simulink model "VFD1"  (R2023b)
settings: Solver=VariableStepAuto  StartTime=0.0  StopTime=6  RelTol=1e-3
libraries: spsACVoltageSourceLib x3, spsSeriesRLCBranchLib x2, spsUniversalBridgeLib x2, spsVoltageMeasurementLib x2, spsAsynchronousMachineSIUnitsLib x1, spsCurrentMeasurementLib x1, spsGroundLib x1, spsIGBTDiodeLib x1, spsPWMGenerator2LevelLib x1, spsRMSLib x1, sps_lib x1
settings Model: Creator=LAB203  LastModifiedBy=LAB203

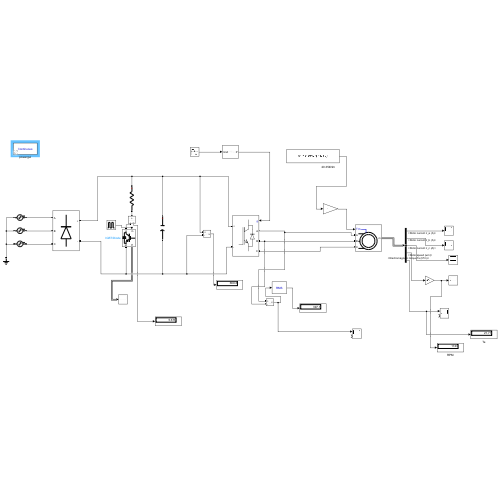
[thumbnail: Simulink's stored preview of the top-level diagram]
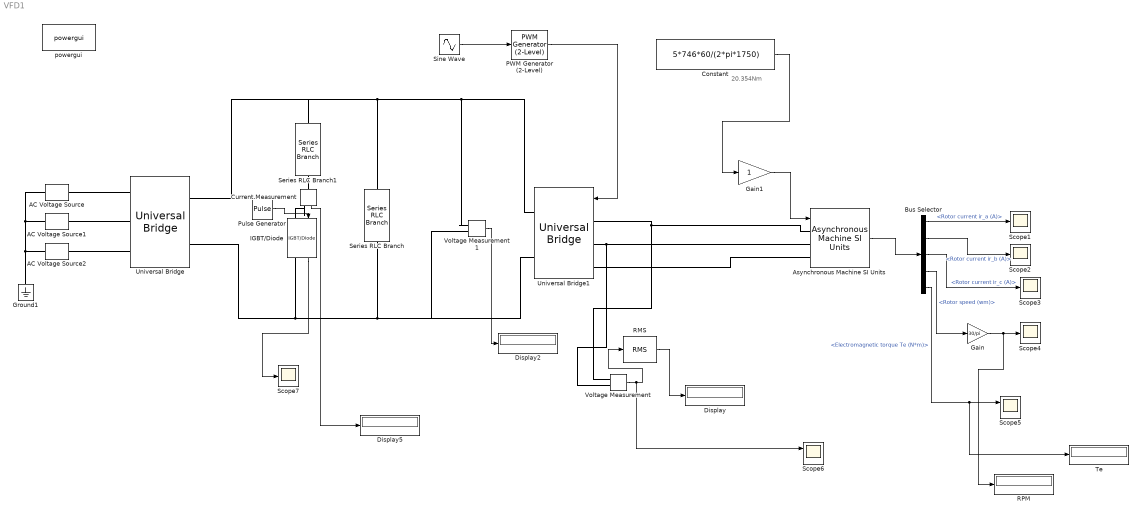
== system VFD1 ==
  note: 20.354Nm
  AC Voltage Source : spsACVoltageSourceLib/AC Voltage Source  Amplitude=400  Phase=0  Frequency=60  SampleTime=0  Measurements=None  BusType=swing  Pref=10e3  Qref=0  Qmin=-inf  Qmax=+inf
  AC Voltage Source1 : spsACVoltageSourceLib/AC Voltage Source  Amplitude=400  Phase=-120  Frequency=60  SampleTime=0  Measurements=None  BusType=swing  Pref=10e3  Qref=0  Qmin=-inf  Qmax=+inf
  AC Voltage Source2 : spsACVoltageSourceLib/AC Voltage Source  Amplitude=400  Phase=120  Frequency=60  SampleTime=0  Measurements=None  BusType=swing  Pref=10e3  Qref=0  Qmin=-inf  Qmax=+inf
  Asynchronous Machine SI Units : spsAsynchronousMachineSIUnitsLib/Asynchronous Machine SI Units  RotorType=Squirrel-cage  PresetModel="01:  5 HP   460 V 60Hz 1750 RPM"  MechanicalLoad=Torque Tm  ShowDetailedParameters=on  ReferenceFrame=Rotor  Units=SI  MeasurementBus=off  NominalParameters=[3730 460 60]  VoltageRatio=1  Stator=[1.115 0.005974]  Rotor=[1.083 0.005974]  Cage1=[0.4155 0.002066]  Cage2=[0.4168 0.0003495]  Lm=0.2037  Mechanical=[0.02 0.005752 2]  PolePairs=2  InitialConditions=[1 0 0 0 0 0 0 0]  SimulateSaturation=off  Saturation=[14.03593122, 27.81365428, 53.79336849, 72.68890987, 97.98006896, 148.6815601, 215.7428561, 302.9841135, 428.7778367 ; 230, 322, 414, 460, 506, 552, 598, 644, 690]  LoadFlowParameters=1492000  TsPowergui=0  TsBlock=-1  IterativeModel=Trapezoidal non iterative  IterativeDiscreteModel=Trapezoidal non iterative  Pmec=3730
  Bus Selector : BusSelector  OutputSignals=Rotor measurements.Rotor current ir_a (A),Rotor measurements.Rotor current ir_b (A),Rotor measurements.Rotor current ir_c (A),Mechanical.Rotor speed (wm),Mechanical.Electromagnetic torque Te (N*m)
  Constant : Constant  Value=5*746*60/(2*pi*1750)
  Current Measurement : spsCurrentMeasurementLib/Current Measurement  PhasorSimulation=off  OutputType=Complex  PSBequivalent=0
  Display : Display
  Display2 : Display
  Display5 : Display
  Gain : Gain  Gain=30/pi
  Gain1 : Gain
  Ground1 : spsGroundLib/Ground  LConnTagsString=a
  IGBT/Diode : spsIGBTDiodeLib/IGBT//Diode  Ron=1e-3  Rs=1e5  Cs=inf  Measurements=on
  PWM Generator (2-Level) : spsPWMGenerator2LevelLib/PWM Generator (2-Level)  ModulatorType=Three-phase bridge (6 pulses)  ModulatorMode=Unsynchronized  Fc=15000  Pc=90  nF=27  MinMax="[ -1.05  1.05 ]"  SamplingTechnique=Natural  ModulatingSignals=off  m=0.85  Freq=60  Phase=0  Ts=0  ShowCarrierOutport=off
  Pulse Generator : DiscretePulseGenerator  PulseType=Time based  Period=10  PulseWidth=50
  RMS : spsRMSLib/RMS  TrueRMS=off  Freq=60  RMSInit=0  Ts=0
  RPM : Display
  Scope{1..4,7} (5 alike) : Scope
  Scope5 : Scope  NumInputPorts=2
  Scope6 : Scope  NumInputPorts=2
  Series RLC Branch : spsSeriesRLCBranchLib/Series RLC Branch  LConnTagsString=__new0  RConnTagsString=__new0  BranchType=C  Resistance=1  Inductance=1e-3  SetiL0=off  InitialCurrent=0  Capacitance=0.881e-3  Setx0=off  InitialVoltage=0  Measurements=None
  Series RLC Branch1 : spsSeriesRLCBranchLib/Series RLC Branch  LConnTagsString=__new0  RConnTagsString=__new0  BranchType=R  Resistance=118  Inductance=1e-3  SetiL0=off  InitialCurrent=0  Capacitance=1e-6  Setx0=off  InitialVoltage=0  Measurements=None
  Sine Wave : Sin  Frequency=2*pi*60  Phase=[0 -2*pi/3 2*pi/3]  SampleTime=0
  Te : Display
  Universal Bridge : spsUniversalBridgeLib/Universal Bridge  Arms=3  SnubberResistance=1e5  SnubberCapacitance=inf  Device=Diodes  Ron=1e-3  Lon=0  ForwardVoltages="[  0  0  ]"  ForwardVoltage=0  GTOparameters=[ 10e-6 , 20e-6 ]  IGBTparameters=[ 1e-6 , 2e-6 ]  Measurements=None  Measurements_2=None  converterType=Rectifier
  Universal Bridge1 : spsUniversalBridgeLib/Universal Bridge  Arms=3  SnubberResistance=1e5  SnubberCapacitance=inf  Device=IGBT / Diodes  Ron=1e-3  Lon=0  ForwardVoltages="[  0  0  ]"  ForwardVoltage=0  GTOparameters=[ 10e-6 , 20e-6 ]  IGBTparameters=[ 1e-6 , 2e-6 ]  Measurements=None  Measurements_2=None  converterType=Rectifier
  Voltage Measurement : spsVoltageMeasurementLib/Voltage Measurement  PhasorSimulation=off  OutputType=Complex  PSBequivalent=0
  Voltage Measurement1 : spsVoltageMeasurementLib/Voltage Measurement  PhasorSimulation=off  OutputType=Complex  PSBequivalent=0
  powergui : sps_lib/powergui  Priority=1  SimulationMode=Continuous  SampleTime=50e-6  frequency=60  Iterations=50  frequencyindice=60  Pbase=100e6  ErrMax=1e-4  UnitsV=kV  UnitsW=MW  buscounter=0  FunctionMessages=off  echomessages=off  EnableUseOfTLC=off  CurrentSourceSwitches=off  DisableSnubberDevices=off  DisableRonSwitches=off  DisableVfSwitches=off  DisplayEquations=off  AutomaticDiscreteSolvers=off  SolverType=Tustin/Backward Euler (TBE)  Interpol=off  ExternalGateDelay=off  methode=off  Ts=100  x0status=blocks  SPID=on  SwTol=0  HookPort=off  NonlinearTolerance=1e-4  nMaxIteration=100  ContinueOnMaxIteration=off  RestoreLinks=warning  ResistiveCurrentMeasurement=off  Frange=[0:2:500]  Ylog=off  Xlog=on  ShowGrid=off  save=off  variable=ZData  structure=0  ZoomFFT=off  StartTime=0.0  cycles=1  DisplayStyle=1  fundamental=60  FreqAxis=off  MaxFrequency=1000  frequencyindicesteady=1  RmsSteady=1  display=off
  wires:
  PWM Generator (2-Level)/1 -> Universal Bridge1/1
  RMS/1 -> Display/1
  Voltage Measurement/1 -> Scope6/1, RMS/1
  Asynchronous Machine SI Units/1 -> Bus Selector/1
  Bus Selector/1 -> Scope1/1  "<Rotor current ir_a (A)>"
  Bus Selector/2 -> Scope2/1  "<Rotor current ir_b (A)>"
  Bus Selector/3 -> Scope3/1  "<Rotor current ir_c (A)>"
  Gain/1 -> RPM/1, Scope4/1
  Bus Selector/4 -> Gain/1  "<Rotor speed (wm)>"
  Bus Selector/5 -> Te/1, Scope5/1  "<Electromagnetic torque Te (N*m)>"
  Constant/1 -> Gain1/1
  Gain1/1 -> Asynchronous Machine SI Units/1
  Voltage Measurement1/1 -> Display2/1
  Pulse Generator/1 -> IGBT/Diode/1
  Current Measurement/1 -> Display5/1
  IGBT/Diode/1 -> Scope7/1
  Sine Wave/1 -> PWM Generator (2-Level)/1
  connections:
  Voltage Measurement1/LConn1 -- Universal Bridge1/RConn1 -- Series RLC Branch/LConn1 -- Universal Bridge/RConn1 -- Series RLC Branch1/LConn1
  Series RLC Branch/RConn1 -- Voltage Measurement1/LConn2 -- Universal Bridge1/RConn2 -- IGBT/Diode/RConn1 -- Universal Bridge/RConn2
  Voltage Measurement/LConn1 -- Asynchronous Machine SI Units/LConn1 -- Universal Bridge1/LConn1
  Voltage Measurement/LConn2 -- Asynchronous Machine SI Units/LConn2 -- Universal Bridge1/LConn2
  AC Voltage Source/RConn1 -- Universal Bridge/LConn1
  AC Voltage Source1/RConn1 -- Universal Bridge/LConn2
  AC Voltage Source2/RConn1 -- Universal Bridge/LConn3
  AC Voltage Source/LConn1 -- AC Voltage Source1/LConn1 -- Ground1/LConn1 -- AC Voltage Source2/LConn1
  Universal Bridge1/LConn3 -- Asynchronous Machine SI Units/LConn3
  Current Measurement/LConn1 -- Series RLC Branch1/RConn1
  Current Measurement/RConn1 -- IGBT/Diode/LConn1
